simulink model "buck"  (R2021a)
settings: Solver=VariableStepAuto  StartTime=0.0  StopTime=10.0  RelTol=1e-3
libraries: spsSeriesRLCBranchLib x3, spsDCVoltageSourceLib x1, spsDiodeLib x1, spsMeanLib x1, spsMosfetLib x1, spsMultimeterLib x1, spspowerguiLib x1
settings Model: Creator=45276  LastModifiedBy=45276

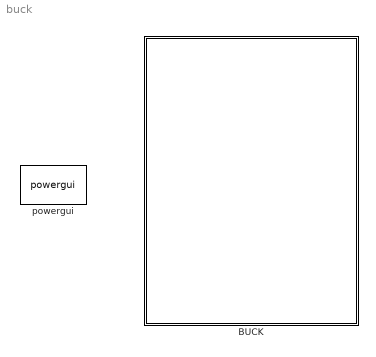
== system buck ==
  BUCK : Subsystem
  powergui : spspowerguiLib/powergui  Priority=1  SimulationMode=Discrete  SampleTime=1e-7  frequency=60  Iterations=50  frequencyindice=0  Pbase=100e6  ErrMax=1e-4  UnitsV=kV  UnitsW=MW  buscounter=0  FunctionMessages=off  echomessages=off  EnableUseOfTLC=off  CurrentSourceSwitches=off  DisableSnubberDevices=off  DisableRonSwitches=off  DisableVfSwitches=off  DisplayEquations=off  AutomaticDiscreteSolvers=off  SolverType=Tustin/Backward Euler (TBE)  Interpol=off  ExternalGateDelay=off  methode=off  Ts=100  x0status=blocks  SPID=off  SwTol=0  HookPort=off  NonlinearTolerance=1e-4  nMaxIteration=100  ContinueOnMaxIteration=off  RestoreLinks=warning  ResistiveCurrentMeasurement=off  Frange=[0:2:500]  Ylog=off  Xlog=on  ShowGrid=off  save=off  variable=ZData  structure=0  ZoomFFT=off  StartTime=0.0  cycles=1  DisplayStyle=1  fundamental=60  FreqAxis=off  MaxFrequency=1000  frequencyindicesteady=1  RmsSteady=1  display=off

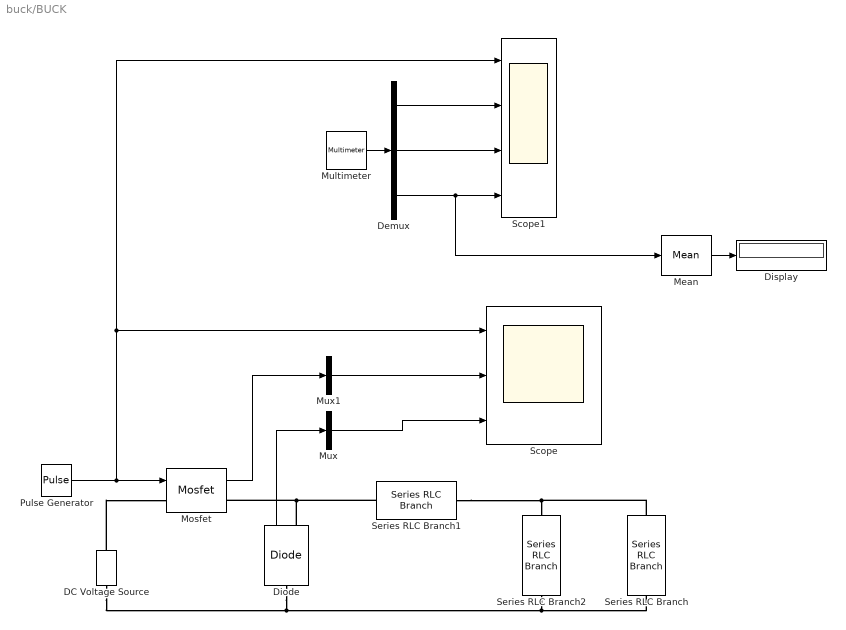
== system buck/BUCK ==
  DC Voltage Source : spsDCVoltageSourceLib/DC Voltage Source  Amplitude=200  Measurements=None
  Demux : Demux  Outputs=3
  Diode : spsDiodeLib/Diode  Ron=0.00000001  Lon=0  Vf=0.8  IC=0  UseSnubber=0  Rs=500  Cs=250e-9  Measurements=on
  Display : Display
  Mean : spsMeanLib/Mean  Freq=60  Vinit=0  Ts=0
  Mosfet : spsMosfetLib/Mosfet  Ron=0.1  Lon=0  Rd=0.01  Vfd=0  IC=0  Rs=1e5  Cs=inf  Measurements=on
  Multimeter : spsMultimeterLib/Multimeter  PhasorSimulation=off  OutputType=Complex  sel=[1 2 3]  L=3  Gain=[1 1 1]  yselected={'Ub: Series RLC Branch','Ub: Series RLC Branch1','Ib: Series RLC Branch1'};  PSBOutputType=1  PSBequivalent=0  AxesSetting=[0,0.1,-100,100]  Display=0  SavedBlockNames=-11
  Mux : Mux  Inputs=1
  Mux1 : Mux  Inputs=1
  Pulse Generator : DiscretePulseGenerator  PulseType=Time based  Period=1/20000  PulseWidth=25
  Scope : Scope  NumInputPorts=3
  Scope1 : Scope  NumInputPorts=4
  Series RLC Branch : spsSeriesRLCBranchLib/Series RLC Branch  LConnTagsString=__new0  RConnTagsString=__new0  BranchType=R  Resistance=20  Inductance=1e-3  SetiL0=off  InitialCurrent=0  Capacitance=1e-6  Setx0=off  InitialVoltage=0  Measurements=Branch voltage
  Series RLC Branch1 : spsSeriesRLCBranchLib/Series RLC Branch  LConnTagsString=__new0  RConnTagsString=__new0  BranchType=L  Resistance=20  Inductance=4.51e-4  SetiL0=off  InitialCurrent=0  Capacitance=1e-6  Setx0=off  InitialVoltage=0  Measurements=Branch voltage and current
  Series RLC Branch2 : spsSeriesRLCBranchLib/Series RLC Branch  LConnTagsString=__new0  RConnTagsString=__new0  BranchType=C  Resistance=20  Inductance=1e-3  SetiL0=off  InitialCurrent=0  Capacitance=2.6e-4  Setx0=off  InitialVoltage=0  Measurements=None
  wires:
  Diode/1 -> Mux/1
  Demux/3 -> Mean/1, Scope1/4
  Demux/2 -> Scope1/3
  Mux1/1 -> Scope/2
  Pulse Generator/1 -> Scope1/1, Scope/1, Mosfet/1
  Demux/1 -> Scope1/2
  Mosfet/1 -> Mux1/1
  Mux/1 -> Scope/3
  Multimeter/1 -> Demux/1
  Mean/1 -> Display/1
  connections:
  DC Voltage Source/LConn1 -- Diode/LConn1 -- Series RLC Branch2/RConn1 -- Series RLC Branch/RConn1
  Series RLC Branch1/RConn1 -- Series RLC Branch/LConn1 -- Series RLC Branch2/LConn1
  Series RLC Branch1/LConn1 -- Diode/RConn1 -- Mosfet/RConn1
  DC Voltage Source/RConn1 -- Mosfet/LConn1
